simulink subsystem "carcomplexsimulink"  (R2025b)
settings: Solver=VariableStepAuto  StartTime=0.0  StopTime=10.0  RelTol=1e-3
settings Model: Creator=sanborkl  LastModifiedBy=sanborkl

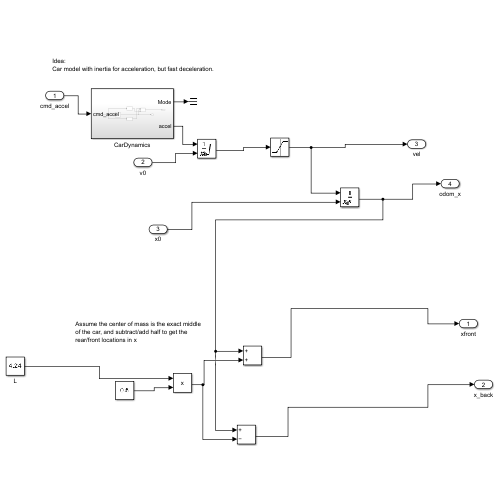
[thumbnail: Simulink's stored preview of the top-level diagram]
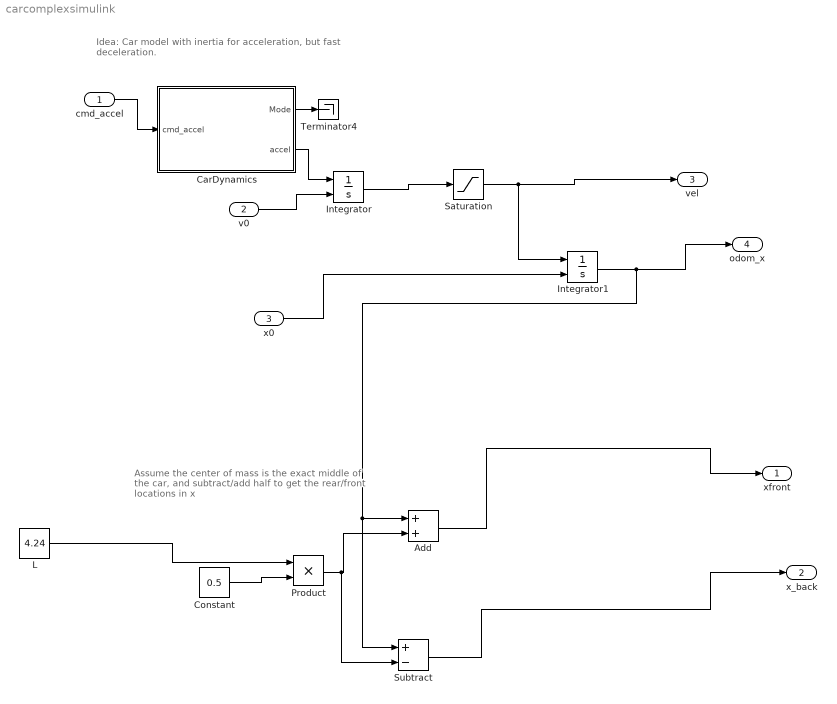
== system carcomplexsimulink ==
  note: Idea:
      | Car model with inertia for acceleration, but fast deceleration.
  note: Assume the center of mass is the exact middle
      | of the car, and subtract/add half to get the
      | rear/front locations in x
  cmd_accel : Inport
  v0 : Inport  Port=2
  x0 : Inport  Port=3
  Add : Sum
  CarDynamics : Subsystem
  Constant : Constant  Value=0.5
  Integrator : Integrator  InitialConditionSource=external  LimitOutput=on  UpperSaturationLimit=40  LowerSaturationLimit=0
  Integrator1 : Integrator  InitialConditionSource=external
  L : Constant  Value=4.24
  Product : Product
  Saturation : Saturate  UpperLimit=40  LowerLimit=0
  Subtract : Sum  Inputs=+-
  Terminator4 : Terminator
  xfront : Outport
  x_back : Outport  Port=2
  vel : Outport  Port=3
  odom_x : Outport  Port=4
  wires:
  Integrator1/1 -> Subtract/1, Add/1, odom_x/1
  CarDynamics/1(Mode) -> Terminator4/1
  Saturation/1 -> Integrator1/1, vel/1
  Add/1 -> xfront/1
  Constant/1 -> Product/2
  Integrator/1 -> Saturation/1
  Subtract/1 -> x_back/1
  Product/1 -> Subtract/2, Add/2
  CarDynamics/2(accel) -> Integrator/1
  cmd_accel/1 -> CarDynamics/1(cmd_accel)
  v0/1 -> Integrator/2
  x0/1 -> Integrator1/2
  L/1 -> Product/1

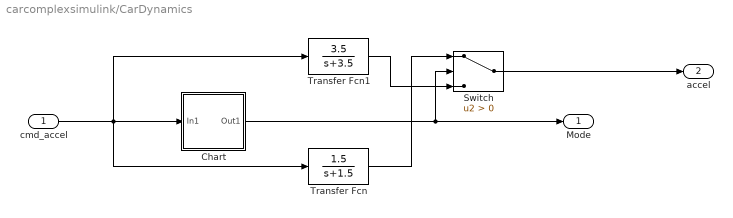
== system carcomplexsimulink/CarDynamics ==
  cmd_accel : Inport
  Chart : Stateflow chart  TreatAsAtomicUnit=on
  Switch : Switch  Criteria=u2 > Threshold  SaturateOnIntegerOverflow=off  InputSameDT=off
  Transfer Fcn : TransferFcn  Numerator=[1.5]  Denominator=[1 1.5]
  Transfer Fcn1 : TransferFcn  Numerator=[3.5]  Denominator=[1 3.5]
  Mode : Outport
  accel : Outport  Port=2
  wires:
  cmd_accel/1 -> Chart/1(In1), Transfer Fcn/1, Transfer Fcn1/1
  Transfer Fcn1/1 -> Switch/3
  Switch/1 -> accel/1
  Transfer Fcn/1 -> Switch/1
  Chart/1(Out1) -> Mode/1, Switch/2

== stateflow chart carcomplexsimulink/CarDynamics/Chart ==
  state Default
    entry: Out1=1;
  state Slowing
    entry: Out1=-1;
  (default) -> Default
  Slowing -> Default : [In1 > 0]
  Default -> Slowing : [In1 < -0.2]
  data: In1 input; Out1 output
